simulink library "casper_library_sources"  (Simulink 8.0)
settings: Solver=ode45  SolverMode=SingleTasking  StartTime=0.0  StopTime=10.0  RelTol=1e-3
values from neighbouring files (symbols this model uses):
  a = [lenba, lenpa, lenta]    [bus_addsub_init.m]    (also in bus_logical_init.m; bus_maddsub_init.m; bus_mult_init.m; bus_relational_init.m)
  b = [lenbb, lenpb, lentb]    [bus_addsub_init.m]    (also in bus_logical_init.m; bus_maddsub_init.m; bus_mult_init.m; bus_relational_init.m)
  quant = 'Round  (unbiased: +/- Inf)'    [bus_addsub_init.m]    (also in bus_convert_init.m = 'Round  (unbiased: Even Values)'; bus_maddsub_init.m; bus_mult_init.m)
undefined symbols (not defined in the file or in its folder): xlipgetpartsetting
libraries: xbsIndex_r4 x11166, casper_library_sources x2
(part 2 of 29)

== system casper_library_sources/Gaussian Random Number Generator/Noise Block 2 ==
  note: The seeds of the individual noise sources can be changed. But the seeds need to be mutually uncorrelated for a particular source
      | i.e. considering only one source say Noise Source -1 ,all the fourteen seeds within that source have to mutually uncorrelated.
  reset : Inport
  Noise Source - 5 : Subsystem  mask(Noise Source Seed Editor){seed1=[0 1 1 0 0 0 0 1 1 1 1 1 1 1 1 0 1 1 1 1 0 1], seed2=[1 0 1 0 1 1 1 1 1 1 0 1 0 1 0 0 1 1 0 1 1 1], seed3=[0 1 1 1 0 1 0 0 0 0 1 1 1 0 0 0 0 1 0 0 0 1], seed4=[1 1 1 0 0 0 0 1 1 0 0 0 1 1 0 0 0 1 0 1 1 0], seed5=[1 0 0 1 0 1 0 1 0 1 1 0 0 1 1 0 1 0 1 0 1 1], seed6=[1 0 1 0 0 0 1 1 0 0 0 1 1 1 0 1 1 0 1 1 0 0], seed7=[0 0 0 0 0 0 1 0 1 1 0 0 1 0 1 0 1 0 0 1 0 0], seed8=[1 1 1 1 0 0 1 0 1 1 0 0 0 1 1 0 1 1 1 0 0 1], seed9=[1 0 0 1 0 0 1 1 1 1 0 1 0 0 0 0 1 0 1 1 1 1], seed10=[0 1 0 1 1 0 1 1 1 1 1 1 1 0 0 0 1 1 0 1 0 1], seed11=[0 1 0 0 0 1 0 1 0 0 1 0 0 0 0 1 1 1 0 1 1 0], seed12=[0 0 0 1 1 0 0 1 0 0 1 0 1 1 0 0 0 0 0 0 0 1], seed13=[1 0 1 1 1 0 1 1 1 0 1 0 0 0 1 0 0 1 1 1 0 1], seed14=[0 1 1 1 1 1 0 0 1 1 0 1 0 0 1 0 1 1 1 0 0 0]}
      mask prompts: seed1 "Seed 1"; seed2 "Seed 2"; seed3 "Seed 3"; seed4 "Seed 4"; seed5 "Seed 5"; seed6 "Seed 6"; seed7 "Seed 7"; seed8 "Seed 8"; seed9 "Seed 9"; seed10 "Seed 10"; seed11 "Seed 11"; seed12 "Seed 12"; seed13 "Seed 13"; seed14 "Seed 14"
      mask help:
      | Please enter the seed of the polynomials for the noise source.
      | Enter the seed as a row matrix of 1s and 0s. Please ensure to
      | have atleast one '1' in each matrix.
  Noise Source - 6 : Subsystem  mask(Noise Source Seed Editor){seed1=[0 1 1 0 1 1 1 1 1 1 0 1 0 1 1 0 1 0 1 1 1 1 0], seed2=[0 0 0 1 0 1 1 0 1 0 0 1 1 0 1 0 1 1 0 0 1 0 0], seed3=[0 0 1 0 1 0 0 0 0 1 0 0 1 1 0 1 1 1 1 1 1 0 0], seed4=[0 1 0 1 1 1 0 1 1 1 0 1 1 1 1 1 0 0 0 1 0 0 0], seed5=[1 0 1 0 1 0 0 1 1 1 1 1 0 1 1 1 0 0 1 1 0 1 0], seed6=[1 0 1 1 1 0 0 0 1 0 0 1 1 1 1 0 0 0 0 1 1 1 0], seed7=[1 0 1 0 0 1 0 1 0 0 1 1 0 0 0 1 1 0 0 0 1 0 0], seed8=[0 1 1 1 1 1 1 1 1 1 1 0 0 0 0 1 0 1 1 1 1 1 1], seed9=[0 1 1 0 0 0 1 0 0 1 0 0 0 1 0 1 1 0 0 0 0 1 1], seed10=[0 0 0 1 0 0 1 0 1 0 1 1 1 1 0 1 1 1 0 1 1 0 1], seed11=[0 0 0 0 0 0 0 1 0 0 0 0 0 1 1 1 0 0 1 0 0 1 0], seed12=[0 0 0 1 0 0 1 1 1 1 1 0 0 1 1 0 1 1 1 0 1 0 1], seed13=[0 0 0 1 0 0 0 1 1 0 0 1 1 1 1 0 0 1 0 1 1 1 1], seed14=[1 0 0 0 0 0 0 1 1 0 1 1 0 0 1 0 1 0 0 1 0 1 0]}
      mask prompts: seed1 "Seed 1"; seed2 "Seed 2"; seed3 "Seed 3"; seed4 "Seed 4"; seed5 "Seed 5"; seed6 "Seed 6"; seed7 "Seed 7"; seed8 "Seed 8"; seed9 "Seed 9"; seed10 "Seed 10"; seed11 "Seed 11"; seed12 "Seed 12"; seed13 "Seed 13"; seed14 "Seed 14"
      mask help:
      | Please enter the seed of the polynomials for the noise source.
      | Enter the seed as a row matrix of 1s and 0s. Please ensure to
      | have atleast one '1' in each matrix.
  Noise Source - 7 : Subsystem  mask(Noise Source Seed Editor){seed1=[1 0 1 0 0 1 0 1 0 1 1 1 0 0 0 1 1 1 1 0 1 1 0 0], seed2=[0 1 1 0 0 1 1 1 1 0 1 1 0 1 1 1 1 0 0 0 0 1 0 0], seed3=[1 1 0 0 0 1 0 1 1 1 0 0 1 1 1 1 0 1 0 0 1 1 0 0], seed4=[0 1 1 0 1 0 0 0 1 0 1 1 0 1 1 0 0 0 0 0 0 1 1 0], seed5=[1 0 0 1 1 1 0 0 1 1 0 0 0 1 0 1 0 0 1 0 0 1 0 1], seed6=[0 1 0 1 0 1 1 1 0 0 0 1 1 0 0 0 0 1 1 1 1 0 1 1], seed7=[1 0 0 1 0 0 1 1 0 0 0 1 0 1 0 1 0 1 0 1 0 0 0 1], seed8=[1 1 1 1 1 1 1 0 1 0 1 1 0 0 0 1 1 1 1 0 1 1 0 1], seed9=[0 1 0 0 0 1 1 1 0 0 0 0 0 1 0 1 1 0 0 1 0 0 1 0], seed10=[1 1 1 1 0 0 0 1 1 1 1 1 1 0 0 0 0 0 0 0 0 0 0 1], seed11=[1 1 1 1 1 0 0 1 0 1 1 1 1 0 1 0 0 0 1 0 0 0 0 1], seed12=[1 0 0 1 0 1 0 1 0 1 1 1 0 1 1 1 1 1 0 0 1 0 0 1], seed13=[1 0 1 1 0 0 1 1 1 1 1 0 0 0 0 0 0 0 0 1 0 0 1 0], seed14=[0 0 1 1 1 0 0 0 1 0 0 0 1 0 1 1 1 1 1 1 1 1 0 1]}
      mask prompts: seed1 "Seed 1"; seed2 "Seed 2"; seed3 "Seed 3"; seed4 "Seed 4"; seed5 "Seed 5"; seed6 "Seed 6"; seed7 "Seed 7"; seed8 "Seed 8"; seed9 "Seed 9"; seed10 "Seed 10"; seed11 "Seed 11"; seed12 "Seed 12"; seed13 "Seed 13"; seed14 "Seed 14"
      mask help:
      | Please enter the seed of the polynomials for the noise source.
      | Enter the seed as a row matrix of 1s and 0s. Please ensure to
      | have atleast one '1' in each matrix.
  Noise Source - 8 : Subsystem  mask(Noise Source Seed Editor){seed1=[0 1 0 1 1 1 0 1 0 1 1 1 1 1 1 0 0 1 1 1 0 0 1 0 1], seed2=[1 0 1 0 1 1 1 1 0 1 0 0 1 1 1 1 1 1 0 1 1 1 0 1 1], seed3=[1 0 1 1 1 0 1 1 1 0 1 1 1 1 1 0 1 0 1 0 1 1 1 1 0], seed4=[1 0 1 0 0 1 1 1 0 1 0 0 0 0 1 0 0 0 0 1 1 1 1 0 1], seed5=[0 0 1 1 0 1 0 0 0 0 1 1 1 0 1 1 0 1 1 0 0 1 1 1 0], seed6=[0 1 1 1 1 0 1 0 0 1 1 0 1 0 1 1 0 1 0 1 0 0 0 0 0], seed7=[0 0 0 0 1 1 1 0 1 0 0 0 1 0 1 0 0 0 0 1 0 0 1 1 1], seed8=[0 1 0 0 0 1 1 0 0 1 0 0 0 0 1 1 1 1 1 0 1 0 0 0 1], seed9=[0 1 0 0 0 1 1 0 1 0 1 0 1 0 0 0 1 1 0 0 0 0 1 1 0], seed10=[0 0 1 0 0 0 1 1 0 1 0 1 0 0 1 1 1 1 0 0 0 0 0 0 0], seed11=[0 1 1 0 1 0 1 1 1 0 1 1 1 0 1 0 1 1 1 0 0 0 1 0 1], seed12=[1 1 0 0 0 1 1 1 0 0 1 0 1 1 0 0 0 1 0 1 1 0 0 1 0], seed13=[0 1 1 1 0 1 1 0 0 0 1 1 0 1 0 1 1 0 0 0 1 0 0 1 0], seed14=[1 0 1 1 1 1 1 1 0 1 0 1 1 1 0 1 0 0 0 0 0 0 1 0 1]}
      mask prompts: seed1 "Seed 1"; seed2 "Seed 2"; seed3 "Seed 3"; seed4 "Seed 4"; seed5 "Seed 5"; seed6 "Seed 6"; seed7 "Seed 7"; seed8 "Seed 8"; seed9 "Seed 9"; seed10 "Seed 10"; seed11 "Seed 11"; seed12 "Seed 12"; seed13 "Seed 13"; seed14 "Seed 14"
      mask help:
      | Please enter the seed of the polynomials for the noise source.
      | Enter the seed as a row matrix of 1s and 0s. Please ensure to
      | have atleast one '1' in each matrix.
  Out1 : Outport
  Out2 : Outport  Port=2
  Out3 : Outport  Port=3
  Out4 : Outport  Port=4
  wires:
  reset/1 -> Noise Source - 8/1(reset), Noise Source - 7/1(reset), Noise Source - 6/1(reset), Noise Source - 5/1(reset)
  Noise Source - 8/1(Out1) -> Out4/1
  Noise Source - 7/1(Out1) -> Out3/1
  Noise Source - 6/1(Out1) -> Out2/1
  Noise Source - 5/1(Out1) -> Out1/1

== system casper_library_sources/tt800_uprng/tt800_engine ==
  note: Delay by (m)
  note: Delay by (n - m - 3)
  seed : Inport
  seed_en : Inport  Port=2
  Constant3 : xbsIndex_r4/Constant  const=0  gui_display_data_type=Fixed-point  arith_type=Unsigned  n_bits=32  bin_pt=0  preci_type=Single  exp_width=8  frac_width=24  explicit_period=off  period=1  equ=P=C  opselect=C  inp2=PCIN>>17  opr=+  inp1=P  carry=CIN  dbl_ovrd=off  block_type=constant
  Gateway Out{1..4} (4 alike) : xbsIndex_r4/Gateway Out  hdl_port=off  timing_constraint=None  locs_specified=off  LOCs={}  block_type=gatewayout
      settings: infoedit="Gateway out block.  Converts Xilinx fixed point inputs into ouputs of type Simulink integer, double, or fixed point.<P><P>Hardware notes:  In hardware these blocks become top level output ports or are discarded, depending on how they are configured."  xl_area=[0 0 0 0 0 0 0]  block_version=10.1.3
  Logical : xbsIndex_r4/Logical  logical_function=XOR  inputs=3  en=off  latency=1  precision=Full  arith_type=Unsigned  n_bits=8  bin_pt=2  align_bp=off  dbl_ovrd=off  block_type=logical
      settings: xl_area=[32 32 0 32 0 0 0]
  Mux : xbsIndex_r4/Mux  inputs=2  en=off  latency=1  precision=Full  arith_type="Signed  (2's comp)"  n_bits=8  bin_pt=2  quantization=Truncate  overflow=Wrap  dbl_ovrd=off  block_type=mux
      settings: xl_area=[16 32 0 32 0 0 0]
  Mux1 : xbsIndex_r4/Mux  inputs=2  en=off  latency=1  precision=Full  arith_type="Signed  (2's comp)"  n_bits=8  bin_pt=2  quantization=Truncate  overflow=Wrap  dbl_ovrd=off  block_type=mux
      settings: xl_area=[16 32 0 32 0 0 0]
  Scope : Scope  NumInputPorts=4
      settings: YMin=-5~-5~-5~-5  YMax=5~5~5~5
  a : xbsIndex_r4/Constant  const=hex2dec('8EBFD028')  gui_display_data_type=Fixed-point  arith_type=Unsigned  n_bits=32  bin_pt=0  preci_type=Single  exp_width=8  frac_width=24  explicit_period=off  period=1  equ=P=C  opselect=C  inp2=PCIN>>17  opr=+  inp1=P  carry=CIN  dbl_ovrd=off  block_type=constant
  delay : xbsIndex_r4/Delay  rst=off  infoeditControl=Selection of Reset will increase slice count due to use of real FFs and instead of SRLs  en=off  latency=1  dbl_ovrd=off  reg_retiming=off  block_type=delay
      settings: xl_area=[16 32 0 0 0 0 0]
  lsb : xbsIndex_r4/Slice  nbits=1  boolean_output=off  mode=Lower Bit Location + Width  bit1=0  base1=MSB of Input  bit0=0  base0=LSB of Input  dbl_ovrd=off  block_type=slice
      settings: infoedit="Extracts a given range of bits from each input sample and presents it at the output.  The output type is ordinarily unsigned with binary point at zero, but can be Boolean when the slice is one bit wide.<P><P>Hardware notes: In hardware this block costs nothing."  block_version=10.1.3
  output : Subsystem
  rshift_1 : xbsIndex_r4/Shift  shift_dir=Right  shift_bits=1  en=off  latency=1  precision=User Defined  arith_type=Unsigned  n_bits=32  bin_pt=0  quantization=Truncate  overflow=Wrap  dbl_ovrd=off  block_type=shift
      settings: xl_area=[0 32 0 0 0 0 0]  block_version=10.1.3
  x_l : xbsIndex_r4/Delay  rst=off  infoeditControl=Selection of Reset will increase slice count due to use of real FFs and instead of SRLs  en=off  latency=7  dbl_ovrd=off  reg_retiming=off  block_type=delay
      settings: xl_area=[16 32 0 32 0 0 0]
  x_l_m : xbsIndex_r4/Delay  rst=off  infoeditControl=Selection of Reset will increase slice count due to use of real FFs and instead of SRLs  en=off  latency=25-7-3  dbl_ovrd=off  reg_retiming=off  block_type=delay
      settings: xl_area=[16 32 0 32 0 0 0]
  u : Outport
  wires:
  x_l_m/1 -> x_l/1, delay/1
  x_l/1 -> lsb/1, rshift_1/1, output/1(in)
  lsb/1 -> Mux/1
  Constant3/1 -> Mux/2
  a/1 -> Mux/3
  rshift_1/1 -> Logical/2
  Mux/1 -> Logical/3
  Logical/1 -> Gateway Out3/1, Mux1/2
  Mux1/1 -> x_l_m/1, Gateway Out2/1
  seed_en/1 -> Gateway Out1/1, Mux1/1
  seed/1 -> Gateway Out4/1, Mux1/3
  Gateway Out1/1 -> Scope/1
  Gateway Out4/1 -> Scope/2
  Gateway Out2/1 -> Scope/3
  Gateway Out3/1 -> Scope/4
  output/1(out) -> u/1
  delay/1 -> Logical/1

== system casper_library_sources/tt800_uprng/tt800_seed_gen ==
  seed_in : Inport
  ld : Inport  Port=2
  Expression : xbsIndex_r4/Expression  expression=(bootstrap | ld | ld_ext)  align_bp=on  en=off  latency=1  precision=Full  arith_type=Unsigned  n_bits=8  bin_pt=2  dbl_ovrd=off  block_type=expr
      settings: xl_area=[0, 0, 0, 0, 0, 0, 0]  block_version=10.1.3
  LFSR : xbsIndex_r4/LFSR  lfsr_type=Fibonacci  gate_type=XOR  n_bits=32  polynomial='C0000401'  rst_value='12345678'  rst=off  en=off  reloadable_seed=on  input_type=on  output_type=on  arith_type=Unsigned  bin_pt=0  dbl_ovrd=off  explicit_period=on  period=1  block_type=lfsr
      settings: xl_area=[17 32 0 33 0 0 0]  block_version=10.1.3
  bootstrap : Subsystem
  p24_extender : Subsystem
  r_edge_detect : Subsystem
  seed_out : Outport
  seed_en : Outport  Port=2
  wires:
  p24_extender/1(out) -> Expression/3
  bootstrap/1(out) -> Expression/1
  LFSR/1 -> seed_out/1
  seed_in/1 -> LFSR/1
  Expression/1 -> seed_en/1
  ld/1 -> Expression/2, r_edge_detect/1(in), LFSR/2
  r_edge_detect/1(out) -> p24_extender/1(in)

== system casper_library_sources/Correlation Control Block/corr_ctrl_blk/NS  26bit ==
  " System Generator" : xbsIndex_r4/ System Generator  Tag=genX  SystemSampleTime=-1  xilinxfamily=virtex5  part=xc5vsx95t  speed=-1  package=ff1136  synthesis_tool=XST  clock_wrapper=Clock Generator(DCM)  directory=./netlist  proj_type=Project Navigator  Synth_file=XST Defaults  Impl_file=ISE Defaults  testbench=off  simulink_period=1  sysclk_period=10  dcm_input_clock_period=100  incr_netlist=off  trim_vbits=Everywhere in SubSystem  dbl_ovrd=According to Block Masks  core_generation=According to Block Masks  run_coregen=off  deprecated_control=off  eval_field=0  block_type=sysgen
      settings: block_version=10.1.3
  AddSub : xbsIndex_r4/AddSub  mode=Subtraction  use_carryin=off  use_carryout=off  en=off  latency=0  precision=User Defined  arith_type="Signed  (2's comp)"  n_bits=8  bin_pt=0  quantization=Truncate  overflow=Wrap  dbl_ovrd=off  use_behavioral_HDL=on  hw_selection=Fabric  pipelined=off  use_rpm=on  block_type=addsub
      settings: xl_area=[0, 0, 0, 0, 0, 0, 0]  block_version=10.1.3
  Adder_Tree : Subsystem
  Constant : xbsIndex_r4/Constant  const=105  gui_display_data_type=Fixed-point  arith_type=Unsigned  n_bits=8  bin_pt=0  preci_type=Single  exp_width=8  frac_width=24  explicit_period=on  period=1  equ=P=C  opselect=C  inp2=PCIN>>17  opr=+  inp1=P  carry=CIN  dbl_ovrd=off  block_type=constant
  Constant1 : xbsIndex_r4/Constant  const=0  gui_display_data_type=Fixed-point  arith_type=Boolean  n_bits=8  bin_pt=0  preci_type=Single  exp_width=8  frac_width=24  explicit_period=on  period=1  equ=P=C  opselect=C  inp2=PCIN>>17  opr=+  inp1=P  carry=CIN  dbl_ovrd=off  block_type=constant
  Resource Estimator : xbsIndex_r4/Resource Estimator  Tag=resEstTag  Slices=0  FFs=0  BRAMs=0  LUTs=0  IOBs=0  EBMs=0  TBUFs=0  xl_use_estimator_area=off  est_options=Estimate  xl_estimator_area=[50 0 0 79 8 0 0]  block_type=resource_estimator
      settings: AttributesFormatString=Resource\nEstimator  block_version=10.1.3
  lfsr_1 : Subsystem  mask{seed=seed1}
  lfsr_10 : Subsystem  mask{seed=seed10}
  lfsr_11 : Subsystem  mask{seed=seed11}
  lfsr_12 : Subsystem  mask{seed=seed12}
  lfsr_13 : Subsystem  mask{seed=seed13}
  lfsr_14 : Subsystem  mask{seed=seed14}
  lfsr_2 : Subsystem  mask{seed=seed2}
  lfsr_3 : Subsystem  mask{seed=seed3}
  lfsr_4 : Subsystem  mask{seed=seed4}
  lfsr_5 : Subsystem  mask{seed=seed5}
  lfsr_6 : Subsystem  mask{seed=seed6}
  lfsr_7 : Subsystem  mask{seed=seed7}
  lfsr_8 : Subsystem  mask{seed=seed8}
  lfsr_9 : Subsystem  mask{seed=seed9}
  Out1 : Outport
  wires:
  lfsr_14/1(Out1) -> Adder_Tree/14(In14)
  lfsr_13/1(Out1) -> Adder_Tree/13(In13)
  lfsr_12/1(Out1) -> Adder_Tree/12(In12)
  lfsr_11/1(Out1) -> Adder_Tree/11(In11)
  lfsr_10/1(Out1) -> Adder_Tree/10(In10)
  lfsr_9/1(Out1) -> Adder_Tree/9(In9)
  lfsr_7/1(Out1) -> Adder_Tree/7(In7)
  lfsr_6/1(Out1) -> Adder_Tree/6(In6)
  lfsr_5/1(Out1) -> Adder_Tree/5(In5)
  lfsr_4/1(Out1) -> Adder_Tree/4(In4)
  lfsr_3/1(Out1) -> Adder_Tree/3(In3)
  lfsr_2/1(Out1) -> Adder_Tree/2(In2)
  AddSub/1 -> Out1/1
  Constant/1 -> AddSub/2
  Adder_Tree/1(Out1) -> AddSub/1
  lfsr_8/1(Out1) -> Adder_Tree/8(In8)
  lfsr_1/1(Out1) -> Adder_Tree/1(In1)
  Constant1/1 -> lfsr_2/1(" reset"), lfsr_3/1(" reset"), lfsr_4/1(" reset"), lfsr_5/1(" reset"), lfsr_6/1(" reset"), lfsr_7/1(" reset"), lfsr_8/1(" reset"), lfsr_9/1(" reset"), lfsr_10/1(" reset"), lfsr_11/1(" reset"), lfsr_12/1(" reset"), lfsr_14/1(" reset"), lfsr_13/1(" reset"), lfsr_1/1(" reset")

== system casper_library_sources/Correlation Control Block/corr_ctrl_blk/NS  27bit ==
  " System Generator" : xbsIndex_r4/ System Generator  Tag=genX  SystemSampleTime=-1  xilinxfamily=virtex5  part=xc5vsx95t  speed=-1  package=ff1136  synthesis_tool=XST  clock_wrapper=Clock Generator(DCM)  directory=./netlist  proj_type=Project Navigator  Synth_file=XST Defaults  Impl_file=ISE Defaults  testbench=off  simulink_period=1  sysclk_period=10  dcm_input_clock_period=100  incr_netlist=off  trim_vbits=Everywhere in SubSystem  dbl_ovrd=According to Block Masks  core_generation=According to Block Masks  run_coregen=off  deprecated_control=off  eval_field=0  block_type=sysgen
      settings: block_version=10.1.3
  AddSub : xbsIndex_r4/AddSub  mode=Subtraction  use_carryin=off  use_carryout=off  en=off  latency=0  precision=User Defined  arith_type="Signed  (2's comp)"  n_bits=8  bin_pt=0  quantization=Truncate  overflow=Wrap  dbl_ovrd=off  use_behavioral_HDL=on  hw_selection=Fabric  pipelined=off  use_rpm=on  block_type=addsub
      settings: xl_area=[0, 0, 0, 0, 0, 0, 0]  block_version=10.1.3
  Adder_Tree : Subsystem
  Constant : xbsIndex_r4/Constant  const=105  gui_display_data_type=Fixed-point  arith_type=Unsigned  n_bits=8  bin_pt=0  preci_type=Single  exp_width=8  frac_width=24  explicit_period=on  period=1  equ=P=C  opselect=C  inp2=PCIN>>17  opr=+  inp1=P  carry=CIN  dbl_ovrd=off  block_type=constant
  Constant1 : xbsIndex_r4/Constant  const=0  gui_display_data_type=Fixed-point  arith_type=Boolean  n_bits=8  bin_pt=0  preci_type=Single  exp_width=8  frac_width=24  explicit_period=on  period=1  equ=P=C  opselect=C  inp2=PCIN>>17  opr=+  inp1=P  carry=CIN  dbl_ovrd=off  block_type=constant
  Resource Estimator : xbsIndex_r4/Resource Estimator  Tag=resEstTag  Slices=0  FFs=0  BRAMs=0  LUTs=0  IOBs=0  EBMs=0  TBUFs=0  xl_use_estimator_area=off  est_options=Estimate  xl_estimator_area=[50 0 0 79 8 0 0]  block_type=resource_estimator
      settings: AttributesFormatString=Resource\nEstimator  block_version=10.1.3
  lfsr_1 : Subsystem  mask{seed=seed1}
  lfsr_10 : Subsystem  mask{seed=seed10}
  lfsr_11 : Subsystem  mask{seed=seed11}
  lfsr_12 : Subsystem  mask{seed=seed12}
  lfsr_13 : Subsystem  mask{seed=seed13}
  lfsr_14 : Subsystem  mask{seed=seed14}
  lfsr_2 : Subsystem  mask{seed=seed2}
  lfsr_3 : Subsystem  mask{seed=seed3}
  lfsr_4 : Subsystem  mask{seed=seed4}
  lfsr_5 : Subsystem  mask{seed=seed5}
  lfsr_6 : Subsystem  mask{seed=seed6}
  lfsr_7 : Subsystem  mask{seed=seed7}
  lfsr_8 : Subsystem  mask{seed=seed8}
  lfsr_9 : Subsystem  mask{seed=seed9}
  Out1 : Outport
  wires:
  lfsr_14/1(Out1) -> Adder_Tree/14(In14)
  lfsr_13/1(Out1) -> Adder_Tree/13(In13)
  lfsr_12/1(Out1) -> Adder_Tree/12(In12)
  lfsr_11/1(Out1) -> Adder_Tree/11(In11)
  lfsr_10/1(Out1) -> Adder_Tree/10(In10)
  lfsr_9/1(Out1) -> Adder_Tree/9(In9)
  lfsr_7/1(Out1) -> Adder_Tree/7(In7)
  lfsr_6/1(Out1) -> Adder_Tree/6(In6)
  lfsr_5/1(Out1) -> Adder_Tree/5(In5)
  lfsr_4/1(Out1) -> Adder_Tree/4(In4)
  lfsr_3/1(Out1) -> Adder_Tree/3(In3)
  lfsr_2/1(Out1) -> Adder_Tree/2(In2)
  AddSub/1 -> Out1/1
  Constant/1 -> AddSub/2
  Adder_Tree/1(Out1) -> AddSub/1
  lfsr_8/1(Out1) -> Adder_Tree/8(In8)
  lfsr_1/1(Out1) -> Adder_Tree/1(In1)
  Constant1/1 -> lfsr_2/1(" reset"), lfsr_3/1(" reset"), lfsr_4/1(" reset"), lfsr_5/1(" reset"), lfsr_6/1(" reset"), lfsr_7/1(" reset"), lfsr_8/1(" reset"), lfsr_9/1(" reset"), lfsr_10/1(" reset"), lfsr_11/1(" reset"), lfsr_12/1(" reset"), lfsr_14/1(" reset"), lfsr_13/1(" reset"), lfsr_1/1(" reset")

== system casper_library_sources/Correlation Control Block/corr_ctrl_blk/NS 28bit ==
  " System Generator" : xbsIndex_r4/ System Generator  Tag=genX  SystemSampleTime=-1  xilinxfamily=virtex5  part=xc5vsx95t  speed=-1  package=ff1136  synthesis_tool=XST  clock_wrapper=Clock Generator(DCM)  directory=./netlist  proj_type=Project Navigator  Synth_file=XST Defaults  Impl_file=ISE Defaults  testbench=off  simulink_period=1  sysclk_period=10  dcm_input_clock_period=100  incr_netlist=off  trim_vbits=Everywhere in SubSystem  dbl_ovrd=According to Block Masks  core_generation=According to Block Masks  run_coregen=off  deprecated_control=off  eval_field=0  block_type=sysgen
      settings: block_version=10.1.3
  AddSub : xbsIndex_r4/AddSub  mode=Subtraction  use_carryin=off  use_carryout=off  en=off  latency=0  precision=User Defined  arith_type="Signed  (2's comp)"  n_bits=8  bin_pt=0  quantization=Truncate  overflow=Wrap  dbl_ovrd=off  use_behavioral_HDL=on  hw_selection=Fabric  pipelined=off  use_rpm=on  block_type=addsub
      settings: xl_area=[0, 0, 0, 0, 0, 0, 0]  block_version=10.1.3
  Adder_Tree : Subsystem
  Constant : xbsIndex_r4/Constant  const=105  gui_display_data_type=Fixed-point  arith_type=Unsigned  n_bits=8  bin_pt=0  preci_type=Single  exp_width=8  frac_width=24  explicit_period=on  period=1  equ=P=C  opselect=C  inp2=PCIN>>17  opr=+  inp1=P  carry=CIN  dbl_ovrd=off  block_type=constant
  Constant1 : xbsIndex_r4/Constant  const=0  gui_display_data_type=Fixed-point  arith_type=Boolean  n_bits=8  bin_pt=0  preci_type=Single  exp_width=8  frac_width=24  explicit_period=on  period=1  equ=P=C  opselect=C  inp2=PCIN>>17  opr=+  inp1=P  carry=CIN  dbl_ovrd=off  block_type=constant
  Resource Estimator : xbsIndex_r4/Resource Estimator  Tag=resEstTag  Slices=0  FFs=0  BRAMs=0  LUTs=0  IOBs=0  EBMs=0  TBUFs=0  xl_use_estimator_area=off  est_options=Estimate  xl_estimator_area=[50 0 0 79 8 0 0]  block_type=resource_estimator
      settings: AttributesFormatString=Resource\nEstimator  block_version=10.1.3
  lfsr_1 : Subsystem  mask{seed=seed1}
  lfsr_10 : Subsystem  mask{seed=seed10}
  lfsr_11 : Subsystem  mask{seed=seed11}
  lfsr_12 : Subsystem  mask{seed=seed12}
  lfsr_13 : Subsystem  mask{seed=seed13}
  lfsr_14 : Subsystem  mask{seed=seed14}
  lfsr_2 : Subsystem  mask{seed=seed2}
  lfsr_3 : Subsystem  mask{seed=seed3}
  lfsr_4 : Subsystem  mask{seed=seed4}
  lfsr_5 : Subsystem  mask{seed=seed5}
  lfsr_6 : Subsystem  mask{seed=seed6}
  lfsr_7 : Subsystem  mask{seed=seed7}
  lfsr_8 : Subsystem  mask{seed=seed8}
  lfsr_9 : Subsystem  mask{seed=seed9}
  Out1 : Outport
  wires:
  lfsr_14/1(Out1) -> Adder_Tree/14(In14)
  lfsr_13/1(Out1) -> Adder_Tree/13(In13)
  lfsr_12/1(Out1) -> Adder_Tree/12(In12)
  lfsr_11/1(Out1) -> Adder_Tree/11(In11)
  lfsr_10/1(Out1) -> Adder_Tree/10(In10)
  lfsr_9/1(Out1) -> Adder_Tree/9(In9)
  lfsr_7/1(Out1) -> Adder_Tree/7(In7)
  lfsr_6/1(Out1) -> Adder_Tree/6(In6)
  lfsr_5/1(Out1) -> Adder_Tree/5(In5)
  lfsr_4/1(Out1) -> Adder_Tree/4(In4)
  lfsr_3/1(Out1) -> Adder_Tree/3(In3)
  lfsr_2/1(Out1) -> Adder_Tree/2(In2)
  AddSub/1 -> Out1/1
  Constant/1 -> AddSub/2
  Adder_Tree/1(Out1) -> AddSub/1
  lfsr_8/1(Out1) -> Adder_Tree/8(In8)
  lfsr_1/1(Out1) -> Adder_Tree/1(In1)
  Constant1/1 -> lfsr_2/1(" reset"), lfsr_3/1(" reset"), lfsr_4/1(" reset"), lfsr_5/1(" reset"), lfsr_6/1(" reset"), lfsr_7/1(" reset"), lfsr_8/1(" reset"), lfsr_9/1(" reset"), lfsr_10/1(" reset"), lfsr_11/1(" reset"), lfsr_12/1(" reset"), lfsr_14/1(" reset"), lfsr_13/1(" reset"), lfsr_1/1(" reset")

== system casper_library_sources/Correlation Control Block/corr_ctrl_blk/NS 29bit ==
  " System Generator" : xbsIndex_r4/ System Generator  Tag=genX  SystemSampleTime=-1  xilinxfamily=virtex5  part=xc5vsx95t  speed=-1  package=ff1136  synthesis_tool=XST  clock_wrapper=Clock Generator(DCM)  directory=./netlist  proj_type=Project Navigator  Synth_file=XST Defaults  Impl_file=ISE Defaults  testbench=off  simulink_period=1  sysclk_period=10  dcm_input_clock_period=100  incr_netlist=off  trim_vbits=Everywhere in SubSystem  dbl_ovrd=According to Block Masks  core_generation=According to Block Masks  run_coregen=off  deprecated_control=off  eval_field=0  block_type=sysgen
      settings: block_version=10.1.3
  AddSub : xbsIndex_r4/AddSub  mode=Subtraction  use_carryin=off  use_carryout=off  en=off  latency=0  precision=User Defined  arith_type="Signed  (2's comp)"  n_bits=8  bin_pt=0  quantization=Truncate  overflow=Wrap  dbl_ovrd=off  use_behavioral_HDL=on  hw_selection=Fabric  pipelined=off  use_rpm=on  block_type=addsub
      settings: xl_area=[0, 0, 0, 0, 0, 0, 0]  block_version=10.1.3
  Adder_Tree : Subsystem
  Constant : xbsIndex_r4/Constant  const=105  gui_display_data_type=Fixed-point  arith_type=Unsigned  n_bits=8  bin_pt=0  preci_type=Single  exp_width=8  frac_width=24  explicit_period=on  period=1  equ=P=C  opselect=C  inp2=PCIN>>17  opr=+  inp1=P  carry=CIN  dbl_ovrd=off  block_type=constant
  Constant1 : xbsIndex_r4/Constant  const=0  gui_display_data_type=Fixed-point  arith_type=Boolean  n_bits=8  bin_pt=0  preci_type=Single  exp_width=8  frac_width=24  explicit_period=on  period=1  equ=P=C  opselect=C  inp2=PCIN>>17  opr=+  inp1=P  carry=CIN  dbl_ovrd=off  block_type=constant
  Resource Estimator : xbsIndex_r4/Resource Estimator  Tag=resEstTag  Slices=0  FFs=0  BRAMs=0  LUTs=0  IOBs=0  EBMs=0  TBUFs=0  xl_use_estimator_area=off  est_options=Estimate  xl_estimator_area=[50 0 0 79 8 0 0]  block_type=resource_estimator
      settings: AttributesFormatString=Resource\nEstimator  block_version=10.1.3
  lfsr_1 : Subsystem  mask{seed=seed1}
  lfsr_10 : Subsystem  mask{seed=seed10}
  lfsr_11 : Subsystem  mask{seed=seed11}
  lfsr_12 : Subsystem  mask{seed=seed12}
  lfsr_13 : Subsystem  mask{seed=seed13}
  lfsr_14 : Subsystem  mask{seed=seed14}
  lfsr_2 : Subsystem  mask{seed=seed2}
  lfsr_3 : Subsystem  mask{seed=seed3}
  lfsr_4 : Subsystem  mask{seed=seed4}
  lfsr_5 : Subsystem  mask{seed=seed5}
  lfsr_6 : Subsystem  mask{seed=seed6}
  lfsr_7 : Subsystem  mask{seed=seed7}
  lfsr_8 : Subsystem  mask{seed=seed8}
  lfsr_9 : Subsystem  mask{seed=seed9}
  Out1 : Outport
  wires:
  lfsr_14/1(Out1) -> Adder_Tree/14(In14)
  lfsr_13/1(Out1) -> Adder_Tree/13(In13)
  lfsr_12/1(Out1) -> Adder_Tree/12(In12)
  lfsr_11/1(Out1) -> Adder_Tree/11(In11)
  lfsr_10/1(Out1) -> Adder_Tree/10(In10)
  lfsr_9/1(Out1) -> Adder_Tree/9(In9)
  lfsr_7/1(Out1) -> Adder_Tree/7(In7)
  lfsr_6/1(Out1) -> Adder_Tree/6(In6)
  lfsr_5/1(Out1) -> Adder_Tree/5(In5)
  lfsr_4/1(Out1) -> Adder_Tree/4(In4)
  lfsr_3/1(Out1) -> Adder_Tree/3(In3)
  lfsr_2/1(Out1) -> Adder_Tree/2(In2)
  AddSub/1 -> Out1/1
  Constant/1 -> AddSub/2
  Adder_Tree/1(Out1) -> AddSub/1
  lfsr_8/1(Out1) -> Adder_Tree/8(In8)
  lfsr_1/1(Out1) -> Adder_Tree/1(In1)
  Constant1/1 -> lfsr_2/1(" reset"), lfsr_3/1(" reset"), lfsr_4/1(" reset"), lfsr_5/1(" reset"), lfsr_6/1(" reset"), lfsr_7/1(" reset"), lfsr_8/1(" reset"), lfsr_9/1(" reset"), lfsr_10/1(" reset"), lfsr_11/1(" reset"), lfsr_12/1(" reset"), lfsr_14/1(" reset"), lfsr_13/1(" reset"), lfsr_1/1(" reset")

== system casper_library_sources/Gaussian Random Number Generator/Noise Block 1/Noise Source - 1 ==
  reset : Inport
  " System Generator" : xbsIndex_r4/ System Generator  Tag=genX  SystemSampleTime=-1  xilinxfamily=virtex5  part=xc5vsx95t  speed=-1  package=ff1136  synthesis_tool=XST  clock_wrapper=Clock Generator(DCM)  directory=./netlist  proj_type=Project Navigator  Synth_file=XST Defaults  Impl_file=ISE Defaults  testbench=off  simulink_period=1  sysclk_period=10  dcm_input_clock_period=100  incr_netlist=off  trim_vbits=Everywhere in SubSystem  dbl_ovrd=According to Block Masks  core_generation=According to Block Masks  run_coregen=off  deprecated_control=off  eval_field=0  block_type=sysgen
      settings: block_version=10.1.3
  AddSub : xbsIndex_r4/AddSub  mode=Subtraction  use_carryin=off  use_carryout=off  en=off  latency=0  precision=User Defined  arith_type="Signed  (2's comp)"  n_bits=8  bin_pt=0  quantization=Truncate  overflow=Wrap  dbl_ovrd=off  use_behavioral_HDL=on  hw_selection=Fabric  pipelined=off  use_rpm=on  block_type=addsub
      settings: xl_area=[0, 0, 0, 0, 0, 0, 0]  block_version=10.1.3
  Adder_Tree : Subsystem
  Constant : xbsIndex_r4/Constant  const=105  gui_display_data_type=Fixed-point  arith_type=Unsigned  n_bits=8  bin_pt=0  preci_type=Single  exp_width=8  frac_width=24  explicit_period=on  period=1  equ=P=C  opselect=C  inp2=PCIN>>17  opr=+  inp1=P  carry=CIN  dbl_ovrd=off  block_type=constant
  Resource Estimator : xbsIndex_r4/Resource Estimator  Tag=resEstTag  Slices=0  FFs=0  BRAMs=0  LUTs=0  IOBs=0  EBMs=0  TBUFs=0  xl_use_estimator_area=off  est_options=Estimate  xl_estimator_area=[50 0 0 79 8 0 0]  block_type=resource_estimator
      settings: AttributesFormatString=Resource\nEstimator  block_version=10.1.3
  lfsr_1 : Subsystem  mask{seed=seed1}
  lfsr_10 : Subsystem  mask{seed=seed10}
  lfsr_11 : Subsystem  mask{seed=seed11}
  lfsr_12 : Subsystem  mask{seed=seed12}
  lfsr_13 : Subsystem  mask{seed=seed13}
  lfsr_14 : Subsystem  mask{seed=seed14}
  lfsr_2 : Subsystem  mask{seed=seed2}
  lfsr_3 : Subsystem  mask{seed=seed3}
  lfsr_4 : Subsystem  mask{seed=seed4}
  lfsr_5 : Subsystem  mask{seed=seed5}
  lfsr_6 : Subsystem  mask{seed=seed6}
  lfsr_7 : Subsystem  mask{seed=seed7}
  lfsr_8 : Subsystem  mask{seed=seed8}
  lfsr_9 : Subsystem  mask{seed=seed9}
  Out1 : Outport
  wires:
  lfsr_14/1(Out1) -> Adder_Tree/14(In14)
  lfsr_13/1(Out1) -> Adder_Tree/13(In13)
  lfsr_12/1(Out1) -> Adder_Tree/12(In12)
  lfsr_11/1(Out1) -> Adder_Tree/11(In11)
  lfsr_10/1(Out1) -> Adder_Tree/10(In10)
  lfsr_9/1(Out1) -> Adder_Tree/9(In9)
  lfsr_7/1(Out1) -> Adder_Tree/7(In7)
  lfsr_6/1(Out1) -> Adder_Tree/6(In6)
  lfsr_5/1(Out1) -> Adder_Tree/5(In5)
  lfsr_4/1(Out1) -> Adder_Tree/4(In4)
  lfsr_3/1(Out1) -> Adder_Tree/3(In3)
  lfsr_2/1(Out1) -> Adder_Tree/2(In2)
  AddSub/1 -> Out1/1
  Constant/1 -> AddSub/2
  Adder_Tree/1(Out1) -> AddSub/1
  lfsr_8/1(Out1) -> Adder_Tree/8(In8)
  lfsr_1/1(Out1) -> Adder_Tree/1(In1)
  reset/1 -> lfsr_7/1(" reset"), lfsr_14/1(" reset"), lfsr_13/1(" reset"), lfsr_12/1(" reset"), lfsr_11/1(" reset"), lfsr_10/1(" reset"), lfsr_9/1(" reset"), lfsr_8/1(" reset"), lfsr_6/1(" reset"), lfsr_5/1(" reset"), lfsr_4/1(" reset"), lfsr_3/1(" reset"), lfsr_2/1(" reset"), lfsr_1/1(" reset")

== system casper_library_sources/Gaussian Random Number Generator/Noise Block 1/Noise Source - 2 ==
  reset : Inport
  " System Generator" : xbsIndex_r4/ System Generator  Tag=genX  SystemSampleTime=-1  xilinxfamily=virtex5  part=xc5vsx95t  speed=-1  package=ff1136  synthesis_tool=XST  clock_wrapper=Clock Generator(DCM)  directory=./netlist  proj_type=Project Navigator  Synth_file=XST Defaults  Impl_file=ISE Defaults  testbench=off  simulink_period=1  sysclk_period=10  dcm_input_clock_period=100  incr_netlist=off  trim_vbits=Everywhere in SubSystem  dbl_ovrd=According to Block Masks  core_generation=According to Block Masks  run_coregen=off  deprecated_control=off  eval_field=0  block_type=sysgen
      settings: block_version=10.1.3
  AddSub : xbsIndex_r4/AddSub  mode=Subtraction  use_carryin=off  use_carryout=off  en=off  latency=0  precision=User Defined  arith_type="Signed  (2's comp)"  n_bits=8  bin_pt=0  quantization=Truncate  overflow=Wrap  dbl_ovrd=off  use_behavioral_HDL=on  hw_selection=Fabric  pipelined=off  use_rpm=on  block_type=addsub
      settings: xl_area=[0, 0, 0, 0, 0, 0, 0]  block_version=10.1.3
  Adder_Tree : Subsystem
  Constant : xbsIndex_r4/Constant  const=105  gui_display_data_type=Fixed-point  arith_type=Unsigned  n_bits=8  bin_pt=0  preci_type=Single  exp_width=8  frac_width=24  explicit_period=on  period=1  equ=P=C  opselect=C  inp2=PCIN>>17  opr=+  inp1=P  carry=CIN  dbl_ovrd=off  block_type=constant
  Resource Estimator : xbsIndex_r4/Resource Estimator  Tag=resEstTag  Slices=0  FFs=0  BRAMs=0  LUTs=0  IOBs=0  EBMs=0  TBUFs=0  xl_use_estimator_area=off  est_options=Estimate  xl_estimator_area=[50 0 0 79 8 0 0]  block_type=resource_estimator
      settings: AttributesFormatString=Resource\nEstimator  block_version=10.1.3
  lfsr_1 : Subsystem  mask{seed=seed1}
  lfsr_10 : Subsystem  mask{seed=seed10}
  lfsr_11 : Subsystem  mask{seed=seed11}
  lfsr_12 : Subsystem  mask{seed=seed12}
  lfsr_13 : Subsystem  mask{seed=seed13}
  lfsr_14 : Subsystem  mask{seed=seed14}
  lfsr_2 : Subsystem  mask{seed=seed2}
  lfsr_3 : Subsystem  mask{seed=seed3}
  lfsr_4 : Subsystem  mask{seed=seed4}
  lfsr_5 : Subsystem  mask{seed=seed5}
  lfsr_6 : Subsystem  mask{seed=seed6}
  lfsr_7 : Subsystem  mask{seed=seed7}
  lfsr_8 : Subsystem  mask{seed=seed8}
  lfsr_9 : Subsystem  mask{seed=seed9}
  Out1 : Outport
  wires:
  lfsr_14/1(Out1) -> Adder_Tree/14(In14)
  lfsr_13/1(Out1) -> Adder_Tree/13(In13)
  lfsr_12/1(Out1) -> Adder_Tree/12(In12)
  lfsr_11/1(Out1) -> Adder_Tree/11(In11)
  lfsr_10/1(Out1) -> Adder_Tree/10(In10)
  lfsr_9/1(Out1) -> Adder_Tree/9(In9)
  lfsr_7/1(Out1) -> Adder_Tree/7(In7)
  lfsr_6/1(Out1) -> Adder_Tree/6(In6)
  lfsr_5/1(Out1) -> Adder_Tree/5(In5)
  lfsr_4/1(Out1) -> Adder_Tree/4(In4)
  lfsr_3/1(Out1) -> Adder_Tree/3(In3)
  lfsr_2/1(Out1) -> Adder_Tree/2(In2)
  AddSub/1 -> Out1/1
  Constant/1 -> AddSub/2
  Adder_Tree/1(Out1) -> AddSub/1
  lfsr_8/1(Out1) -> Adder_Tree/8(In8)
  lfsr_1/1(Out1) -> Adder_Tree/1(In1)
  reset/1 -> lfsr_2/1(" reset"), lfsr_3/1(" reset"), lfsr_4/1(" reset"), lfsr_5/1(" reset"), lfsr_6/1(" reset"), lfsr_7/1(" reset"), lfsr_8/1(" reset"), lfsr_9/1(" reset"), lfsr_10/1(" reset"), lfsr_11/1(" reset"), lfsr_12/1(" reset"), lfsr_14/1(" reset"), lfsr_13/1(" reset"), lfsr_1/1(" reset")

== system casper_library_sources/Gaussian Random Number Generator/Noise Block 1/Noise Source - 3 ==
  reset : Inport
  " System Generator" : xbsIndex_r4/ System Generator  Tag=genX  SystemSampleTime=-1  xilinxfamily=virtex5  part=xc5vsx95t  speed=-1  package=ff1136  synthesis_tool=XST  clock_wrapper=Clock Generator(DCM)  directory=./netlist  proj_type=Project Navigator  Synth_file=XST Defaults  Impl_file=ISE Defaults  testbench=off  simulink_period=1  sysclk_period=10  dcm_input_clock_period=100  incr_netlist=off  trim_vbits=Everywhere in SubSystem  dbl_ovrd=According to Block Masks  core_generation=According to Block Masks  run_coregen=off  deprecated_control=off  eval_field=0  block_type=sysgen
      settings: block_version=10.1.3
  AddSub : xbsIndex_r4/AddSub  mode=Subtraction  use_carryin=off  use_carryout=off  en=off  latency=0  precision=User Defined  arith_type="Signed  (2's comp)"  n_bits=8  bin_pt=0  quantization=Truncate  overflow=Wrap  dbl_ovrd=off  use_behavioral_HDL=on  hw_selection=Fabric  pipelined=off  use_rpm=on  block_type=addsub
      settings: xl_area=[0, 0, 0, 0, 0, 0, 0]  block_version=10.1.3
  Adder_Tree : Subsystem
  Constant : xbsIndex_r4/Constant  const=105  gui_display_data_type=Fixed-point  arith_type=Unsigned  n_bits=8  bin_pt=0  preci_type=Single  exp_width=8  frac_width=24  explicit_period=on  period=1  equ=P=C  opselect=C  inp2=PCIN>>17  opr=+  inp1=P  carry=CIN  dbl_ovrd=off  block_type=constant
  Resource Estimator : xbsIndex_r4/Resource Estimator  Tag=resEstTag  Slices=0  FFs=0  BRAMs=0  LUTs=0  IOBs=0  EBMs=0  TBUFs=0  xl_use_estimator_area=off  est_options=Estimate  xl_estimator_area=[50 0 0 79 8 0 0]  block_type=resource_estimator
      settings: AttributesFormatString=Resource\nEstimator  block_version=10.1.3
  lfsr_1 : Subsystem  mask{seed=seed1}
  lfsr_10 : Subsystem  mask{seed=seed10}
  lfsr_11 : Subsystem  mask{seed=seed11}
  lfsr_12 : Subsystem  mask{seed=seed12}
  lfsr_13 : Subsystem  mask{seed=seed13}
  lfsr_14 : Subsystem  mask{seed=seed14}
  lfsr_2 : Subsystem  mask{seed=seed2}
  lfsr_3 : Subsystem  mask{seed=seed3}
  lfsr_4 : Subsystem  mask{seed=seed4}
  lfsr_5 : Subsystem  mask{seed=seed5}
  lfsr_6 : Subsystem  mask{seed=seed6}
  lfsr_7 : Subsystem  mask{seed=seed7}
  lfsr_8 : Subsystem  mask{seed=seed8}
  lfsr_9 : Subsystem  mask{seed=seed9}
  Out1 : Outport
  wires:
  lfsr_14/1(Out1) -> Adder_Tree/14(In14)
  lfsr_13/1(Out1) -> Adder_Tree/13(In13)
  lfsr_12/1(Out1) -> Adder_Tree/12(In12)
  lfsr_11/1(Out1) -> Adder_Tree/11(In11)
  lfsr_10/1(Out1) -> Adder_Tree/10(In10)
  lfsr_9/1(Out1) -> Adder_Tree/9(In9)
  lfsr_7/1(Out1) -> Adder_Tree/7(In7)
  lfsr_6/1(Out1) -> Adder_Tree/6(In6)
  lfsr_5/1(Out1) -> Adder_Tree/5(In5)
  lfsr_4/1(Out1) -> Adder_Tree/4(In4)
  lfsr_3/1(Out1) -> Adder_Tree/3(In3)
  lfsr_2/1(Out1) -> Adder_Tree/2(In2)
  AddSub/1 -> Out1/1
  Constant/1 -> AddSub/2
  Adder_Tree/1(Out1) -> AddSub/1
  lfsr_8/1(Out1) -> Adder_Tree/8(In8)
  lfsr_1/1(Out1) -> Adder_Tree/1(In1)
  reset/1 -> lfsr_2/1(" reset"), lfsr_3/1(" reset"), lfsr_4/1(" reset"), lfsr_5/1(" reset"), lfsr_6/1(" reset"), lfsr_7/1(" reset"), lfsr_8/1(" reset"), lfsr_9/1(" reset"), lfsr_10/1(" reset"), lfsr_11/1(" reset"), lfsr_12/1(" reset"), lfsr_14/1(" reset"), lfsr_13/1(" reset"), lfsr_1/1(" reset")

== system casper_library_sources/Gaussian Random Number Generator/Noise Block 1/Noise Source - 4 ==
  reset : Inport
  " System Generator" : xbsIndex_r4/ System Generator  Tag=genX  SystemSampleTime=-1  xilinxfamily=virtex5  part=xc5vsx95t  speed=-1  package=ff1136  synthesis_tool=XST  clock_wrapper=Clock Generator(DCM)  directory=./netlist  proj_type=Project Navigator  Synth_file=XST Defaults  Impl_file=ISE Defaults  testbench=off  simulink_period=1  sysclk_period=10  dcm_input_clock_period=100  incr_netlist=off  trim_vbits=Everywhere in SubSystem  dbl_ovrd=According to Block Masks  core_generation=According to Block Masks  run_coregen=off  deprecated_control=off  eval_field=0  block_type=sysgen
      settings: block_version=10.1.3
  AddSub : xbsIndex_r4/AddSub  mode=Subtraction  use_carryin=off  use_carryout=off  en=off  latency=0  precision=User Defined  arith_type="Signed  (2's comp)"  n_bits=8  bin_pt=0  quantization=Truncate  overflow=Wrap  dbl_ovrd=off  use_behavioral_HDL=on  hw_selection=Fabric  pipelined=off  use_rpm=on  block_type=addsub
      settings: xl_area=[0, 0, 0, 0, 0, 0, 0]  block_version=10.1.3
  Adder_Tree : Subsystem
  Constant : xbsIndex_r4/Constant  const=105  gui_display_data_type=Fixed-point  arith_type=Unsigned  n_bits=8  bin_pt=0  preci_type=Single  exp_width=8  frac_width=24  explicit_period=on  period=1  equ=P=C  opselect=C  inp2=PCIN>>17  opr=+  inp1=P  carry=CIN  dbl_ovrd=off  block_type=constant
  Resource Estimator : xbsIndex_r4/Resource Estimator  Tag=resEstTag  Slices=0  FFs=0  BRAMs=0  LUTs=0  IOBs=0  EBMs=0  TBUFs=0  xl_use_estimator_area=off  est_options=Estimate  xl_estimator_area=[50 0 0 79 8 0 0]  block_type=resource_estimator
      settings: AttributesFormatString=Resource\nEstimator  block_version=10.1.3
  lfsr_1 : Subsystem  mask{seed=seed1}
  lfsr_10 : Subsystem  mask{seed=seed10}
  lfsr_11 : Subsystem  mask{seed=seed11}
  lfsr_12 : Subsystem  mask{seed=seed12}
  lfsr_13 : Subsystem  mask{seed=seed13}
  lfsr_14 : Subsystem  mask{seed=seed14}
  lfsr_2 : Subsystem  mask{seed=seed2}
  lfsr_3 : Subsystem  mask{seed=seed3}
  lfsr_4 : Subsystem  mask{seed=seed4}
  lfsr_5 : Subsystem  mask{seed=seed5}
  lfsr_6 : Subsystem  mask{seed=seed6}
  lfsr_7 : Subsystem  mask{seed=seed7}
  lfsr_8 : Subsystem  mask{seed=seed8}
  lfsr_9 : Subsystem  mask{seed=seed9}
  Out1 : Outport
  wires:
  lfsr_14/1(Out1) -> Adder_Tree/14(In14)
  lfsr_13/1(Out1) -> Adder_Tree/13(In13)
  lfsr_12/1(Out1) -> Adder_Tree/12(In12)
  lfsr_11/1(Out1) -> Adder_Tree/11(In11)
  lfsr_10/1(Out1) -> Adder_Tree/10(In10)
  lfsr_9/1(Out1) -> Adder_Tree/9(In9)
  lfsr_7/1(Out1) -> Adder_Tree/7(In7)
  lfsr_6/1(Out1) -> Adder_Tree/6(In6)
  lfsr_5/1(Out1) -> Adder_Tree/5(In5)
  lfsr_4/1(Out1) -> Adder_Tree/4(In4)
  lfsr_3/1(Out1) -> Adder_Tree/3(In3)
  lfsr_2/1(Out1) -> Adder_Tree/2(In2)
  AddSub/1 -> Out1/1
  Constant/1 -> AddSub/2
  Adder_Tree/1(Out1) -> AddSub/1
  lfsr_8/1(Out1) -> Adder_Tree/8(In8)
  lfsr_1/1(Out1) -> Adder_Tree/1(In1)
  reset/1 -> lfsr_2/1(" reset"), lfsr_3/1(" reset"), lfsr_4/1(" reset"), lfsr_5/1(" reset"), lfsr_6/1(" reset"), lfsr_7/1(" reset"), lfsr_8/1(" reset"), lfsr_9/1(" reset"), lfsr_10/1(" reset"), lfsr_11/1(" reset"), lfsr_12/1(" reset"), lfsr_14/1(" reset"), lfsr_13/1(" reset"), lfsr_1/1(" reset")

== system casper_library_sources/Gaussian Random Number Generator/Noise Block 2/Noise Source - 5 ==
  reset : Inport
  " System Generator" : xbsIndex_r4/ System Generator  Tag=genX  SystemSampleTime=-1  xilinxfamily=virtex5  part=xc5vsx95t  speed=-1  package=ff1136  synthesis_tool=XST  clock_wrapper=Clock Generator(DCM)  directory=./netlist  proj_type=Project Navigator  Synth_file=XST Defaults  Impl_file=ISE Defaults  testbench=off  simulink_period=1  sysclk_period=10  dcm_input_clock_period=100  incr_netlist=off  trim_vbits=Everywhere in SubSystem  dbl_ovrd=According to Block Masks  core_generation=According to Block Masks  run_coregen=off  deprecated_control=off  eval_field=0  block_type=sysgen
      settings: block_version=10.1.3
  AddSub : xbsIndex_r4/AddSub  mode=Subtraction  use_carryin=off  use_carryout=off  en=off  latency=0  precision=User Defined  arith_type="Signed  (2's comp)"  n_bits=8  bin_pt=0  quantization=Truncate  overflow=Wrap  dbl_ovrd=off  use_behavioral_HDL=on  hw_selection=Fabric  pipelined=off  use_rpm=on  block_type=addsub
      settings: xl_area=[0, 0, 0, 0, 0, 0, 0]  block_version=10.1.3
  Adder_Tree : Subsystem
  Constant : xbsIndex_r4/Constant  const=105  gui_display_data_type=Fixed-point  arith_type=Unsigned  n_bits=8  bin_pt=0  preci_type=Single  exp_width=8  frac_width=24  explicit_period=on  period=1  equ=P=C  opselect=C  inp2=PCIN>>17  opr=+  inp1=P  carry=CIN  dbl_ovrd=off  block_type=constant
  Resource Estimator : xbsIndex_r4/Resource Estimator  Tag=resEstTag  Slices=0  FFs=0  BRAMs=0  LUTs=0  IOBs=0  EBMs=0  TBUFs=0  xl_use_estimator_area=off  est_options=Estimate  xl_estimator_area=[50 0 0 79 8 0 0]  block_type=resource_estimator
      settings: AttributesFormatString=Resource\nEstimator  block_version=10.1.3
  lfsr_1 : Subsystem  mask{seed=seed1}
  lfsr_10 : Subsystem  mask{seed=seed10}
  lfsr_11 : Subsystem  mask{seed=seed11}
  lfsr_12 : Subsystem  mask{seed=seed12}
  lfsr_13 : Subsystem  mask{seed=seed13}
  lfsr_14 : Subsystem  mask{seed=seed14}
  lfsr_2 : Subsystem  mask{seed=seed2}
  lfsr_3 : Subsystem  mask{seed=seed3}
  lfsr_4 : Subsystem  mask{seed=seed4}
  lfsr_5 : Subsystem  mask{seed=seed5}
  lfsr_6 : Subsystem  mask{seed=seed6}
  lfsr_7 : Subsystem  mask{seed=seed7}
  lfsr_8 : Subsystem  mask{seed=seed8}
  lfsr_9 : Subsystem  mask{seed=seed9}
  Out1 : Outport
  wires:
  lfsr_14/1(Out1) -> Adder_Tree/14(In14)
  lfsr_13/1(Out1) -> Adder_Tree/13(In13)
  lfsr_12/1(Out1) -> Adder_Tree/12(In12)
  lfsr_11/1(Out1) -> Adder_Tree/11(In11)
  lfsr_10/1(Out1) -> Adder_Tree/10(In10)
  lfsr_9/1(Out1) -> Adder_Tree/9(In9)
  lfsr_7/1(Out1) -> Adder_Tree/7(In7)
  lfsr_6/1(Out1) -> Adder_Tree/6(In6)
  lfsr_5/1(Out1) -> Adder_Tree/5(In5)
  lfsr_4/1(Out1) -> Adder_Tree/4(In4)
  lfsr_3/1(Out1) -> Adder_Tree/3(In3)
  lfsr_2/1(Out1) -> Adder_Tree/2(In2)
  AddSub/1 -> Out1/1
  Constant/1 -> AddSub/2
  Adder_Tree/1(Out1) -> AddSub/1
  lfsr_8/1(Out1) -> Adder_Tree/8(In8)
  lfsr_1/1(Out1) -> Adder_Tree/1(In1)
  reset/1 -> lfsr_2/1(" reset"), lfsr_3/1(" reset"), lfsr_4/1(" reset"), lfsr_5/1(" reset"), lfsr_6/1(" reset"), lfsr_7/1(" reset"), lfsr_8/1(" reset"), lfsr_9/1(" reset"), lfsr_10/1(" reset"), lfsr_11/1(" reset"), lfsr_12/1(" reset"), lfsr_14/1(" reset"), lfsr_13/1(" reset"), lfsr_1/1(" reset")

== system casper_library_sources/Gaussian Random Number Generator/Noise Block 2/Noise Source - 6 ==
  reset : Inport
  " System Generator" : xbsIndex_r4/ System Generator  Tag=genX  SystemSampleTime=-1  xilinxfamily=virtex5  part=xc5vsx95t  speed=-1  package=ff1136  synthesis_tool=XST  clock_wrapper=Clock Generator(DCM)  directory=./netlist  proj_type=Project Navigator  Synth_file=XST Defaults  Impl_file=ISE Defaults  testbench=off  simulink_period=1  sysclk_period=10  dcm_input_clock_period=100  incr_netlist=off  trim_vbits=Everywhere in SubSystem  dbl_ovrd=According to Block Masks  core_generation=According to Block Masks  run_coregen=off  deprecated_control=off  eval_field=0  block_type=sysgen
      settings: block_version=10.1.3
  AddSub : xbsIndex_r4/AddSub  mode=Subtraction  use_carryin=off  use_carryout=off  en=off  latency=0  precision=User Defined  arith_type="Signed  (2's comp)"  n_bits=8  bin_pt=0  quantization=Truncate  overflow=Wrap  dbl_ovrd=off  use_behavioral_HDL=on  hw_selection=Fabric  pipelined=off  use_rpm=on  block_type=addsub
      settings: xl_area=[0, 0, 0, 0, 0, 0, 0]  block_version=10.1.3
  Adder_Tree : Subsystem
  Constant : xbsIndex_r4/Constant  const=105  gui_display_data_type=Fixed-point  arith_type=Unsigned  n_bits=8  bin_pt=0  preci_type=Single  exp_width=8  frac_width=24  explicit_period=on  period=1  equ=P=C  opselect=C  inp2=PCIN>>17  opr=+  inp1=P  carry=CIN  dbl_ovrd=off  block_type=constant
  Resource Estimator : xbsIndex_r4/Resource Estimator  Tag=resEstTag  Slices=0  FFs=0  BRAMs=0  LUTs=0  IOBs=0  EBMs=0  TBUFs=0  xl_use_estimator_area=off  est_options=Estimate  xl_estimator_area=[50 0 0 79 8 0 0]  block_type=resource_estimator
      settings: AttributesFormatString=Resource\nEstimator  block_version=10.1.3
  lfsr_1 : Subsystem  mask{seed=seed1}
  lfsr_10 : Subsystem  mask{seed=seed10}
  lfsr_11 : Subsystem  mask{seed=seed11}
  lfsr_12 : Subsystem  mask{seed=seed12}
  lfsr_13 : Subsystem  mask{seed=seed13}
  lfsr_14 : Subsystem  mask{seed=seed14}
  lfsr_2 : Subsystem  mask{seed=seed2}
  lfsr_3 : Subsystem  mask{seed=seed3}
  lfsr_4 : Subsystem  mask{seed=seed4}
  lfsr_5 : Subsystem  mask{seed=seed5}
  lfsr_6 : Subsystem  mask{seed=seed6}
  lfsr_7 : Subsystem  mask{seed=seed7}
  lfsr_8 : Subsystem  mask{seed=seed8}
  lfsr_9 : Subsystem  mask{seed=seed9}
  Out1 : Outport
  wires:
  lfsr_14/1(Out1) -> Adder_Tree/14(In14)
  lfsr_13/1(Out1) -> Adder_Tree/13(In13)
  lfsr_12/1(Out1) -> Adder_Tree/12(In12)
  lfsr_11/1(Out1) -> Adder_Tree/11(In11)
  lfsr_10/1(Out1) -> Adder_Tree/10(In10)
  lfsr_9/1(Out1) -> Adder_Tree/9(In9)
  lfsr_7/1(Out1) -> Adder_Tree/7(In7)
  lfsr_6/1(Out1) -> Adder_Tree/6(In6)
  lfsr_5/1(Out1) -> Adder_Tree/5(In5)
  lfsr_4/1(Out1) -> Adder_Tree/4(In4)
  lfsr_3/1(Out1) -> Adder_Tree/3(In3)
  lfsr_2/1(Out1) -> Adder_Tree/2(In2)
  AddSub/1 -> Out1/1
  Constant/1 -> AddSub/2
  Adder_Tree/1(Out1) -> AddSub/1
  lfsr_8/1(Out1) -> Adder_Tree/8(In8)
  lfsr_1/1(Out1) -> Adder_Tree/1(In1)
  reset/1 -> lfsr_2/1(" reset"), lfsr_3/1(" reset"), lfsr_4/1(" reset"), lfsr_5/1(" reset"), lfsr_6/1(" reset"), lfsr_7/1(" reset"), lfsr_8/1(" reset"), lfsr_9/1(" reset"), lfsr_10/1(" reset"), lfsr_11/1(" reset"), lfsr_12/1(" reset"), lfsr_14/1(" reset"), lfsr_13/1(" reset"), lfsr_1/1(" reset")

== system casper_library_sources/Gaussian Random Number Generator/Noise Block 2/Noise Source - 7 ==
  reset : Inport
  " System Generator" : xbsIndex_r4/ System Generator  Tag=genX  SystemSampleTime=-1  xilinxfamily=virtex5  part=xc5vsx95t  speed=-1  package=ff1136  synthesis_tool=XST  clock_wrapper=Clock Generator(DCM)  directory=./netlist  proj_type=Project Navigator  Synth_file=XST Defaults  Impl_file=ISE Defaults  testbench=off  simulink_period=1  sysclk_period=10  dcm_input_clock_period=100  incr_netlist=off  trim_vbits=Everywhere in SubSystem  dbl_ovrd=According to Block Masks  core_generation=According to Block Masks  run_coregen=off  deprecated_control=off  eval_field=0  block_type=sysgen
      settings: block_version=10.1.3
  AddSub : xbsIndex_r4/AddSub  mode=Subtraction  use_carryin=off  use_carryout=off  en=off  latency=0  precision=User Defined  arith_type="Signed  (2's comp)"  n_bits=8  bin_pt=0  quantization=Truncate  overflow=Wrap  dbl_ovrd=off  use_behavioral_HDL=on  hw_selection=Fabric  pipelined=off  use_rpm=on  block_type=addsub
      settings: xl_area=[0, 0, 0, 0, 0, 0, 0]  block_version=10.1.3
  Adder_Tree : Subsystem
  Constant : xbsIndex_r4/Constant  const=105  gui_display_data_type=Fixed-point  arith_type=Unsigned  n_bits=8  bin_pt=0  preci_type=Single  exp_width=8  frac_width=24  explicit_period=on  period=1  equ=P=C  opselect=C  inp2=PCIN>>17  opr=+  inp1=P  carry=CIN  dbl_ovrd=off  block_type=constant
  Resource Estimator : xbsIndex_r4/Resource Estimator  Tag=resEstTag  Slices=0  FFs=0  BRAMs=0  LUTs=0  IOBs=0  EBMs=0  TBUFs=0  xl_use_estimator_area=off  est_options=Estimate  xl_estimator_area=[50 0 0 79 8 0 0]  block_type=resource_estimator
      settings: AttributesFormatString=Resource\nEstimator  block_version=10.1.3
  lfsr_1 : Subsystem  mask{seed=seed1}
  lfsr_10 : Subsystem  mask{seed=seed10}
  lfsr_11 : Subsystem  mask{seed=seed11}
  lfsr_12 : Subsystem  mask{seed=seed12}
  lfsr_13 : Subsystem  mask{seed=seed13}
  lfsr_14 : Subsystem  mask{seed=seed14}
  lfsr_2 : Subsystem  mask{seed=seed2}
  lfsr_3 : Subsystem  mask{seed=seed3}
  lfsr_4 : Subsystem  mask{seed=seed4}
  lfsr_5 : Subsystem  mask{seed=seed5}
  lfsr_6 : Subsystem  mask{seed=seed6}
  lfsr_7 : Subsystem  mask{seed=seed7}
  lfsr_8 : Subsystem  mask{seed=seed8}
  lfsr_9 : Subsystem  mask{seed=seed9}
  Out1 : Outport
  wires:
  lfsr_14/1(Out1) -> Adder_Tree/14(In14)
  lfsr_13/1(Out1) -> Adder_Tree/13(In13)
  lfsr_12/1(Out1) -> Adder_Tree/12(In12)
  lfsr_11/1(Out1) -> Adder_Tree/11(In11)
  lfsr_10/1(Out1) -> Adder_Tree/10(In10)
  lfsr_9/1(Out1) -> Adder_Tree/9(In9)
  lfsr_7/1(Out1) -> Adder_Tree/7(In7)
  lfsr_6/1(Out1) -> Adder_Tree/6(In6)
  lfsr_5/1(Out1) -> Adder_Tree/5(In5)
  lfsr_4/1(Out1) -> Adder_Tree/4(In4)
  lfsr_3/1(Out1) -> Adder_Tree/3(In3)
  lfsr_2/1(Out1) -> Adder_Tree/2(In2)
  AddSub/1 -> Out1/1
  Constant/1 -> AddSub/2
  Adder_Tree/1(Out1) -> AddSub/1
  lfsr_8/1(Out1) -> Adder_Tree/8(In8)
  lfsr_1/1(Out1) -> Adder_Tree/1(In1)
  reset/1 -> lfsr_2/1(" reset"), lfsr_3/1(" reset"), lfsr_4/1(" reset"), lfsr_5/1(" reset"), lfsr_6/1(" reset"), lfsr_7/1(" reset"), lfsr_8/1(" reset"), lfsr_9/1(" reset"), lfsr_10/1(" reset"), lfsr_11/1(" reset"), lfsr_12/1(" reset"), lfsr_14/1(" reset"), lfsr_13/1(" reset"), lfsr_1/1(" reset")
